simulink model "Assignment_1"  (R2026a)
settings: Solver=VariableStepAuto  StopTime=60
values from neighbouring files (symbols this model uses):
  a = 1    [Assignment_1_param.m]
  a_m = 2    [Assignment_1_param.m]
  b = 2    [Assignment_1_param.m]
libraries: simulink x2
settings Model: Creator=saradenti  LastModifiedBy=saradenti

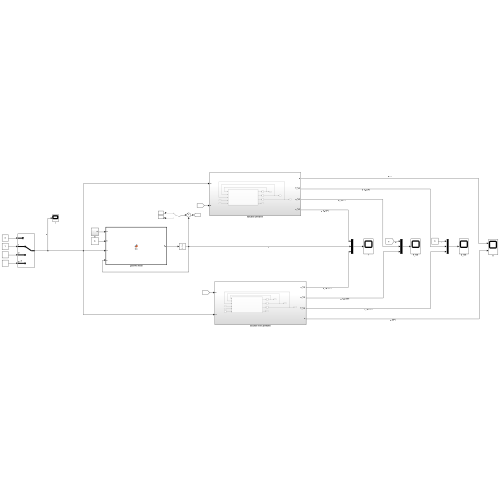
[thumbnail: Simulink's stored preview of the top-level diagram]
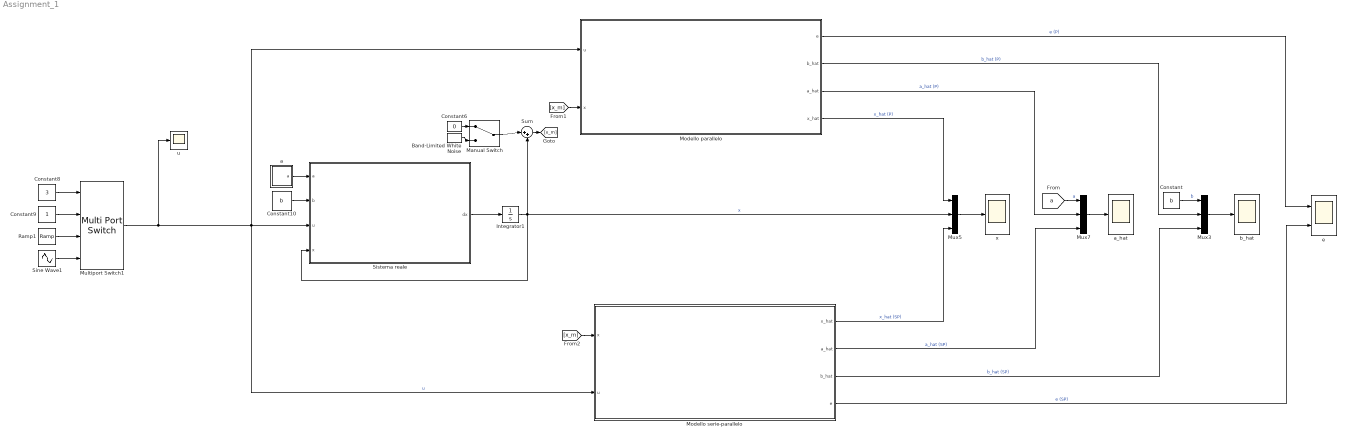
== system Assignment_1 ==
  Band-Limited White Noise : simulink/Sources/Band-Limited White Noise  Cov=[0.1]  Ts=0.1  seed=[23341]
  Constant : Constant  Value=b
  Constant10 : Constant  Value=b
  Constant6 : Constant  Value=0
  Constant8 : Constant  Value=3
  Constant9 : Constant
  Integrator1 : Integrator
  Manual Switch : ManualSwitch
  Modello parallelo : Subsystem
  Modello serie-parallelo : Subsystem
  Multiport Switch1 : MultiPortSwitch  SaturateOnIntegerOverflow=off  InputSameDT=off
  Mux3 : Mux  Inputs=3
  Mux5 : Mux  Inputs=3
  Mux7 : Mux  Inputs=3
  Ramp1 : simulink/Sources/Ramp  slope=1  start=0  InitialOutput=0
  Sine Wave1 : Sin  SampleTime=0
  Sistema reale : MATLAB Function  TreatAsAtomicUnit=on
  Sum : Sum  Inputs=|++
  a : Subsystem
  a_hat : Scope
      settings: ActiveDisplayYMinimum=-0.52867916695433548  ActiveDisplayYMaximum=1.1703380529154537  DataLoggingVariableName=ScopeData5
  b_hat : Scope
      settings: ActiveDisplayYMinimum=-4.0230761232688135  ActiveDisplayYMaximum=3.9195027094109793  DataLoggingVariableName=ScopeData6
  e : Scope  NumInputPorts=2
      settings: ActiveDisplayYMinimum=-1.2569668920604735  ActiveDisplayYMaximum=1.1863279407014076  DataLoggingVariableName=ScopeData10
  u : Scope
      settings: ActiveDisplayYMinimum=-1.2499882002266689  ActiveDisplayYMaximum=1.2499917365329862  DataLoggingVariableName=ScopeData9
  x : Scope
      settings: ActiveDisplayYMinimum=-2.0330510305351495  ActiveDisplayYMaximum=2.3062618874019445  DataLoggingVariableName=ScopeData8
  wires:
  Constant8/1 -> Multiport Switch1/1
  Integrator1/1 -> Sistema reale/4(x), Sum/2, Mux5/2  "x"
  Constant9/1 -> Multiport Switch1/2
  Sine Wave1/1 -> Multiport Switch1/4
  Ramp1/1 -> Multiport Switch1/3
  Constant10/1 -> Sistema reale/2(b)
  Modello parallelo/1(e) -> e/1  "e (P)"
  Modello parallelo/3(a_hat) -> Mux7/2  "a_hat (P)"
  Modello parallelo/2(b_hat) -> Mux3/2  "b_hat (P)"
  Sistema reale/1(dx) -> Integrator1/1
  Mux5/1 -> x/1
  Multiport Switch1/1 -> u/1, Modello parallelo/1(u), Sistema reale/3(u), Modello serie-parallelo/2(u)  "u"
  Modello parallelo/4(x_hat) -> Mux5/1  "x_hat (P)"
  Modello serie-parallelo/1(x_hat) -> Mux5/3  "x_hat (SP)"
  a/1(a) -> Sistema reale/1(a)
  Modello serie-parallelo/4(e) -> e/2  "e (SP)"
  Modello serie-parallelo/2(a_hat) -> Mux7/3  "a_hat (SP)"
  Mux3/1 -> b_hat/1
  Modello serie-parallelo/3(b_hat) -> Mux3/3  "b_hat (SP)"
  Mux7/1 -> a_hat/1
  [a] -> Mux7/1  "a"
  Constant/1 -> Mux3/1  "b"
  Manual Switch/1 -> Sum/1
  Sum/1 -> [x_m]
  [x_m] -> Modello parallelo/2(x)
  [x_m] -> Modello serie-parallelo/1(x)
  Band-Limited White Noise/1 -> Manual Switch/2
  Constant6/1 -> Manual Switch/1

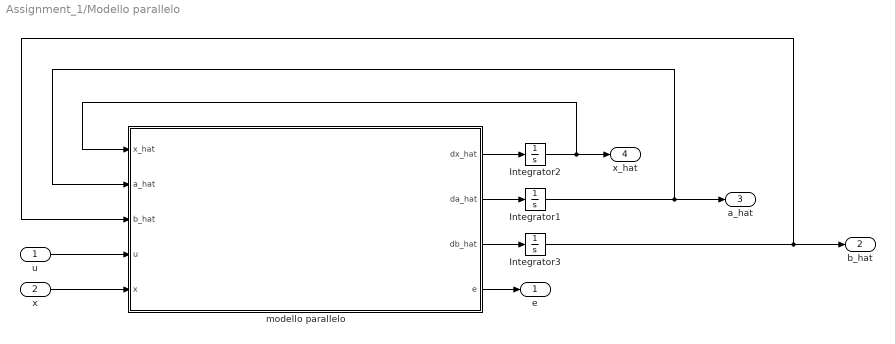
== system Assignment_1/Modello parallelo ==
  u : Inport
  x : Inport  Port=2
  Integrator1 : Integrator
  Integrator2 : Integrator
  Integrator3 : Integrator
  modello parallelo : MATLAB Function  TreatAsAtomicUnit=on
  e : Outport
  b_hat : Outport  Port=2
  a_hat : Outport  Port=3
  x_hat : Outport  Port=4
  wires:
  u/1 -> modello parallelo/4(u)
  x/1 -> modello parallelo/5(x)
  modello parallelo/1(dx_hat) -> Integrator2/1
  modello parallelo/2(da_hat) -> Integrator1/1
  Integrator1/1 -> modello parallelo/2(a_hat), a_hat/1
  modello parallelo/3(db_hat) -> Integrator3/1
  Integrator3/1 -> b_hat/1, modello parallelo/3(b_hat)
  Integrator2/1 -> x_hat/1, modello parallelo/1(x_hat)
  modello parallelo/4(e) -> e/1

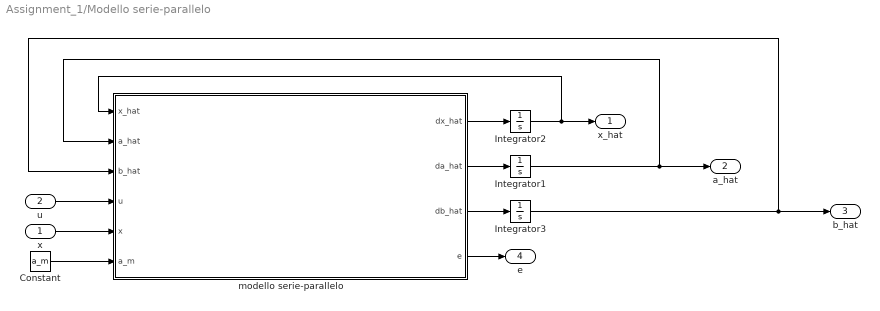
== system Assignment_1/Modello serie-parallelo ==
  x : Inport
  u : Inport  Port=2
  Constant : Constant  Value=a_m
  Integrator1 : Integrator
  Integrator2 : Integrator
  Integrator3 : Integrator
  modello serie-parallelo : MATLAB Function  TreatAsAtomicUnit=on
  x_hat : Outport
  a_hat : Outport  Port=2
  b_hat : Outport  Port=3
  e : Outport  Port=4
  wires:
  u/1 -> modello serie-parallelo/4(u)
  x/1 -> modello serie-parallelo/5(x)
  modello serie-parallelo/1(dx_hat) -> Integrator2/1
  modello serie-parallelo/2(da_hat) -> Integrator1/1
  Integrator1/1 -> modello serie-parallelo/2(a_hat), a_hat/1
  modello serie-parallelo/3(db_hat) -> Integrator3/1
  Integrator3/1 -> b_hat/1, modello serie-parallelo/3(b_hat)
  Integrator2/1 -> x_hat/1, modello serie-parallelo/1(x_hat)
  modello serie-parallelo/4(e) -> e/1
  Constant/1 -> modello serie-parallelo/6(a_m)

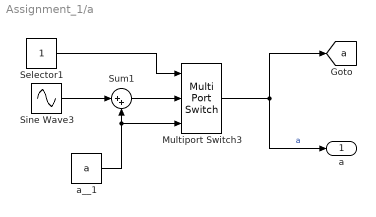
== system Assignment_1/a ==
  Multiport Switch3 : MultiPortSwitch  Inputs=2  SaturateOnIntegerOverflow=off  InputSameDT=off
  Selector1 : Constant
  Sine Wave3 : Sin  Amplitude=0.1  Frequency=2*pi/(24*3600)  SampleTime=0
  Sum1 : Sum  Inputs=|++
  a__1 : Constant  Value=a
  a : Outport
  tag scope: a=global
  wires:
  Multiport Switch3/1 -> [a], a/1  "a"
  Sum1/1 -> Multiport Switch3/2
  a__1/1 -> Multiport Switch3/3, Sum1/2
  Selector1/1 -> Multiport Switch3/1
  Sine Wave3/1 -> Sum1/1

== matlab function Assignment_1/Sistema reale ==
  data: a input; b input; u input; x input; dx output
function dx = fcn(a,b,u,x)


    dx= -a*x+b*u;

== matlab function Assignment_1/Modello parallelo/modello parallelo ==
  data: dx_hat output; da_hat output; db_hat output; x_hat input; a_hat input; b_hat input; u input; x input; e output
function [dx_hat,da_hat,db_hat,e] = fcn(x_hat,a_hat,b_hat,u,x)

    e = x_hat - x;

    dx_hat = - a_hat * x_hat + b_hat * u;
    
    da_hat = x_hat * e;

    db_hat = - e * u;

== matlab function Assignment_1/Modello serie-parallelo/modello serie-parallelo ==
  data: dx_hat output; da_hat output; db_hat output; x_hat input; a_hat input; b_hat input; u input; x input; e output; a_m input
function [dx_hat,da_hat,db_hat,e] = fcn(x_hat,a_hat,b_hat,u,x, a_m)

    e = x_hat - x;

    dx_hat = - a_m * x_hat + (a_m - a_hat) * x + b_hat * u;
    
    da_hat = x * e;

    db_hat = - e * u;
